simulink model "Ideal_2ndOrder_PI_Sat_CtlStep"  (R2013b)
settings: Solver=ode45  StartTime=0.0  StopTime=sim_stop_time  FixedStep=sim_step_size  MaxStep=sim_step_size  RelTol=1e-3
PreLoadFcn:
  | motor_parameters;
values from neighbouring files (symbols this model uses):
  b = 0.0006001689451    [Ideal_2ndOrder_PI_Prop_only.mat]    (also in Ideal_2ndOrder_PI_Sat.mat; Ideal_2ndOrder_PI_Sat_CtlStep.mat; Ideal_2ndOrder_PI_Sat_CtlStep_Q.mat; Ideal_2ndOrder_PI_Sat_CtlStep_Q_verification.mat)
  ctl_step_size = 0.03    [Ideal_2ndOrder_PI_Sat_CtlStep.mat]    (also in Ideal_2ndOrder_PI_Sat_CtlStep_Q.mat; Ideal_2ndOrder_PI_Sat_CtlStep_Q_verification.mat; Ideal_2ndOrder_PI_Sat_CtlStep_Q_verify_deploy.mat = 0.01; Ideal_PI_Sat_CtlStep_Q_run.m)
  J = 0.001321184025    [Ideal_2ndOrder_PI_Prop_only.mat]    (also in Ideal_2ndOrder_PI_Sat.mat; Ideal_2ndOrder_PI_Sat_CtlStep.mat; Ideal_2ndOrder_PI_Sat_CtlStep_Q.mat; Ideal_2ndOrder_PI_Sat_CtlStep_Q_verification.mat)
  Kb = 0.4952900056    [Ideal_2ndOrder_PI_Prop_only.mat]    (also in Ideal_2ndOrder_PI_Sat.mat; Ideal_2ndOrder_PI_Sat_CtlStep.mat; Ideal_2ndOrder_PI_Sat_CtlStep_Q.mat; Ideal_2ndOrder_PI_Sat_CtlStep_Q_verification.mat)
  Ki = 0    [Ideal_2ndOrder_PI_Prop_only.mat]    (also in Ideal_2ndOrder_PI_Sat.mat = 38; Ideal_2ndOrder_PI_Sat_CtlStep.mat = 38; Ideal_2ndOrder_PI_Sat_CtlStep_Q.mat = 38; Ideal_2ndOrder_PI_Sat_CtlStep_Q_verification.mat = 38)
  Kp = 0.9    [Ideal_2ndOrder_PI_Prop_only.mat]    (also in Ideal_2ndOrder_PI_Sat.mat; Ideal_2ndOrder_PI_Sat_CtlStep.mat; Ideal_2ndOrder_PI_Sat_CtlStep_Q.mat; Ideal_2ndOrder_PI_Sat_CtlStep_Q_verification.mat)
  Kt = 0.3233728703    [Ideal_2ndOrder_PI_Prop_only.mat]    (also in Ideal_2ndOrder_PI_Sat.mat; Ideal_2ndOrder_PI_Sat_CtlStep.mat; Ideal_2ndOrder_PI_Sat_CtlStep_Q.mat; Ideal_2ndOrder_PI_Sat_CtlStep_Q_verification.mat)
  L = 0.0047    [Ideal_2ndOrder_PI_Prop_only.mat]    (also in Ideal_2ndOrder_PI_Sat.mat; Ideal_2ndOrder_PI_Sat_CtlStep.mat; Ideal_2ndOrder_PI_Sat_CtlStep_Q.mat; Ideal_2ndOrder_PI_Sat_CtlStep_Q_verification.mat)
  LoopGain = 1    [Ideal_2ndOrder_PI_Sat.mat]    (also in Ideal_2ndOrder_PI_Sat_CtlStep.mat = 0.15; Ideal_2ndOrder_PI_Sat_CtlStep_Q.mat = 0.12; Ideal_2ndOrder_PI_Sat_CtlStep_Q_verification.mat = 0.12; Ideal_2ndOrder_PI_Sat_CtlStep_Q_verify_deploy.mat = 0.12)
  R = 5.262773292    [Ideal_2ndOrder_PI_Prop_only.mat]    (also in Ideal_2ndOrder_PI_Sat.mat; Ideal_2ndOrder_PI_Sat_CtlStep.mat; Ideal_2ndOrder_PI_Sat_CtlStep_Q.mat; Ideal_2ndOrder_PI_Sat_CtlStep_Q_verification.mat)
  sim_step_size = 0.0001    [Ideal_2ndOrder_PI_Prop_only.mat]    (also in Ideal_2ndOrder_PI_Sat.mat; Ideal_2ndOrder_PI_Sat_CtlStep.mat; Ideal_2ndOrder_PI_Sat_CtlStep_Q.mat; Ideal_2ndOrder_PI_Sat_CtlStep_Q_verification.mat = 0.01)
  Veloref = 12    [Ideal_2ndOrder_PI_Prop_only.mat]    (also in Ideal_2ndOrder_PI_Sat.mat; Ideal_2ndOrder_PI_Sat_CtlStep.mat; Ideal_2ndOrder_PI_Sat_CtlStep_Q.mat; Ideal_2ndOrder_PI_Sat_CtlStep_Q_verification.mat = 3.14)
  Vref = 9    [Ideal_2ndOrder_PI_Prop_only.mat]    (also in Ideal_2ndOrder_PI_Sat.mat; Ideal_2ndOrder_PI_Sat_CtlStep.mat; Ideal_2ndOrder_PI_Sat_CtlStep_Q.mat; Ideal_2ndOrder_PI_Sat_CtlStep_Q_verification.mat = 4.5)
libraries: simulink x1
settings Model: Creator=nding  LastModifiedBy=nding

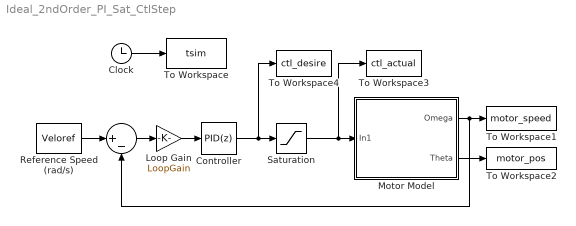
== system Ideal_2ndOrder_PI_Sat_CtlStep ==
  " " : Sum  Inputs=|+-
  Clock : Clock
  Controller : simulink/Continuous/PID Controller  Controller=PID  TimeDomain=Discrete-time  SampleTime=ctl_step_size  IntegratorMethod=Forward Euler  FilterMethod=Forward Euler  Form=Parallel  P=Kp  I=Ki  D=0  N=100  InitialConditionSource=internal  InitialConditionForIntegrator=0  InitialConditionForFilter=0  ExternalReset=none  LimitOutput=off  UpperSaturationLimit=inf  LowerSaturationLimit=-inf  LinearizeAsGain=off  AntiWindupMode=none  Kb=1  TrackingMode=off  Kt=1  PParamMin=[]  PParamMax=[]  IParamMin=[]  IParamMax=[]  DParamMin=[]  DParamMax=[]  NParamMin=[]  NParamMax=[]  KbParamMin=[]  KbParamMax=[]  KtParamMin=[]  KtParamMax=[]  POutMin=[]  POutMax=[]  IOutMin=[]  IOutMax=[]  DOutMin=[]  DOutMax=[]  NOutMin=[]  NOutMax=[]  KbOutMin=[]  KbOutMax=[]  KtOutMin=[]  KtOutMax=[]  IntegratorOutMin=[]  IntegratorOutMax=[]  FilterOutMin=[]  FilterOutMax=[]  SumOutMin=[]  SumOutMax=[]  SumI1OutMin=[]  SumI1OutMax=[]  SumI2OutMin=[]  SumI2OutMax=[]  SumI3OutMin=[]  SumI3OutMax=[]  SumDOutMin=[]  SumDOutMax=[]  SaturationOutMin=[]  SaturationOutMax=[]  IntegratorContinuousStateAttributes=''  IntegratorStateMustResolveToSignalObject=off  IntegratorRTWStateStorageClass=Auto  FilterContinuousStateAttributes=''  FilterStateMustResolveToSignalObject=off  FilterRTWStateStorageClass=Auto
  Loop Gain : Gain  Gain=LoopGain
  Motor Model : Subsystem
  Reference Speed (rad/s) : Constant  Value=Veloref
  Saturation : Saturate  UpperLimit=Vref  LowerLimit=-Vref
  To Workspace : ToWorkspace  VariableName=tsim  SampleTime=sim_step_size
  To Workspace1 : ToWorkspace  VariableName=motor_speed  SampleTime=sim_step_size
  To Workspace2 : ToWorkspace  VariableName=motor_pos  SampleTime=sim_step_size
  To Workspace3 : ToWorkspace  VariableName=ctl_actual  SampleTime=sim_step_size
  To Workspace4 : ToWorkspace  VariableName=ctl_desire  SampleTime=sim_step_size
  wires:
  Clock/1 -> To Workspace/1
  Motor Model/1(Omega) -> " "/2, To Workspace1/1
  Motor Model/2(Theta) -> To Workspace2/1
  Reference Speed (rad/s)/1 -> " "/1
  Controller/1 -> To Workspace4/1, Saturation/1
  Loop Gain/1 -> Controller/1
  " "/1 -> Loop Gain/1
  Saturation/1 -> To Workspace3/1, Motor Model/1(In1)

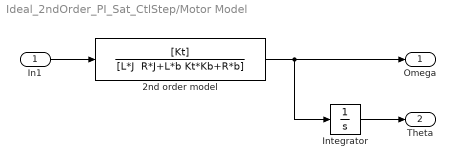
== system Ideal_2ndOrder_PI_Sat_CtlStep/Motor Model ==
  In1 : Inport
  2nd order model : TransferFcn  Numerator=[Kt]  Denominator="[L*J  R*J+L*b Kt*Kb+R*b]"
  Integrator : Integrator
  Omega : Outport
  Theta : Outport  Port=2
  wires:
  2nd order model/1 -> Omega/1, Integrator/1
  In1/1 -> 2nd order model/1
  Integrator/1 -> Theta/1
